simulink model "implfb_can_unpack"  (R2026b)
settings: Solver=VariableStepAuto
undefined symbols (not defined in the file or in its folder): Ts
libraries: simulink x4, svdutilitieslib x1
settings Model: Creator=aomar  LastModifiedBy=aomar

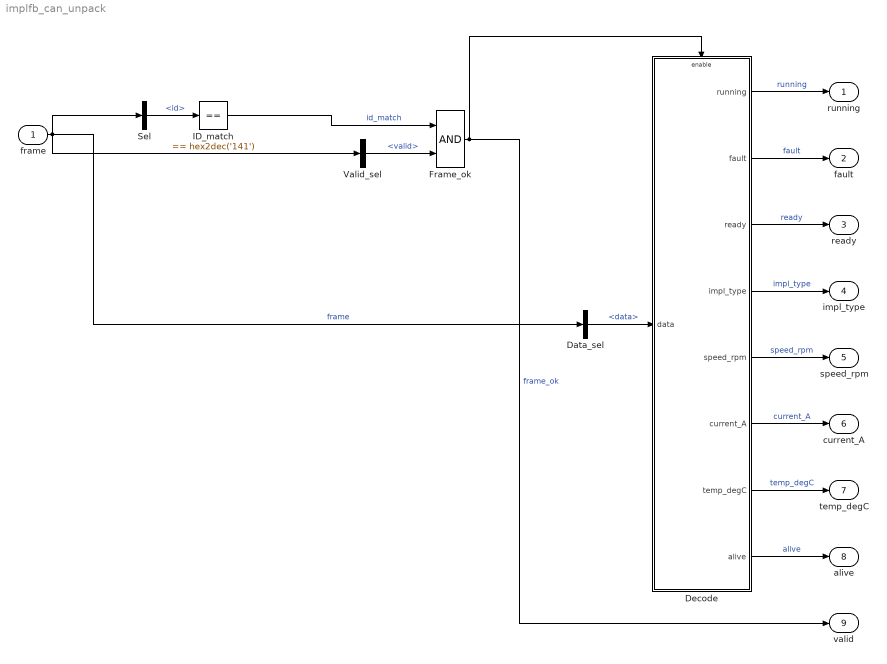
== system implfb_can_unpack ==
  frame : Inport  OutDataTypeStr=Bus: Bus_CanFrame8  SampleTime=Ts.can_slow
  Data_sel : BusSelector  OutputSignals=data
  Decode : Subsystem  TreatAsAtomicUnit=on
  Frame_ok : Logic  AllPortsSameDT=off  OutDataTypeStr=boolean
  ID_match : simulink/Logic and Bit Operations/Compare To Constant  relop===  const=hex2dec('141')  OutDataTypeStr=boolean
  Sel : BusSelector  OutputSignals=id
  Valid_sel : BusSelector  OutputSignals=valid
  running : Outport
  fault : Outport  Port=2
  ready : Outport  Port=3
  impl_type : Outport  Port=4
  speed_rpm : Outport  Port=5
  current_A : Outport  Port=6
  temp_degC : Outport  Port=7
  alive : Outport  Port=8
  valid : Outport  Port=9  OutDataTypeStr=boolean
  wires:
  frame/1 -> Data_sel/1, Sel/1, Valid_sel/1  "frame"
  Sel/1 -> ID_match/1  "<id>"
  ID_match/1 -> Frame_ok/1  "id_match"
  Valid_sel/1 -> Frame_ok/2  "<valid>"
  Frame_ok/1 -> valid/1, Decode/Enable  "frame_ok"
  Data_sel/1 -> Decode/1(data)  "<data>"
  Decode/1(running) -> running/1  "running"
  Decode/2(fault) -> fault/1  "fault"
  Decode/3(ready) -> ready/1  "ready"
  Decode/4(impl_type) -> impl_type/1  "impl_type"
  Decode/5(speed_rpm) -> speed_rpm/1  "speed_rpm"
  Decode/6(current_A) -> current_A/1  "current_A"
  Decode/7(temp_degC) -> temp_degC/1  "temp_degC"
  Decode/8(alive) -> alive/1  "alive"

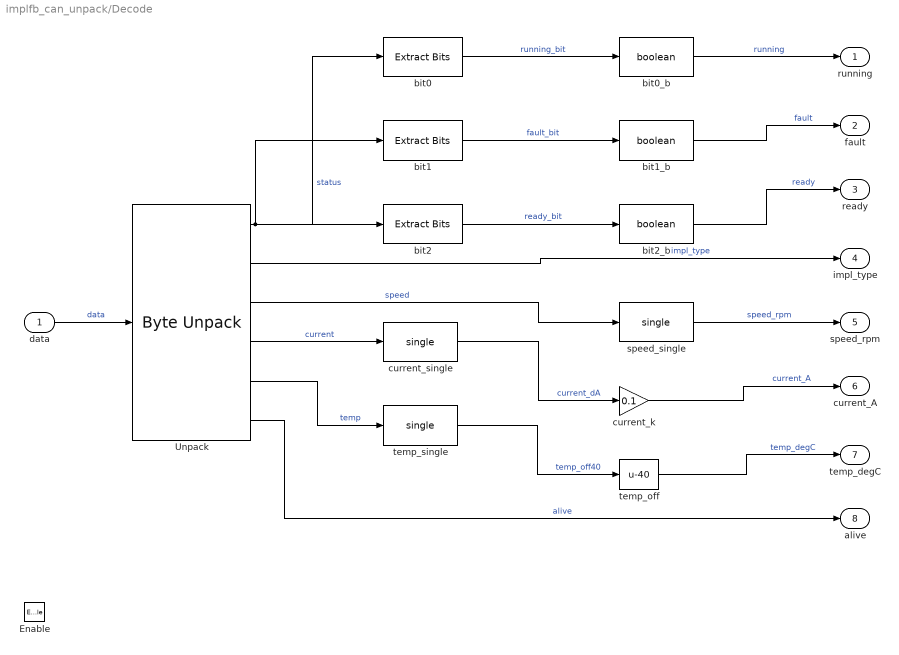
== system implfb_can_unpack/Decode ==
  data : Inport
  Enable : EnablePort
  Unpack : svdutilitieslib/Byte Unpack  dimensions={1,1,1,1,1,1}  datatypes={'uint8','uint8','int16','int16','uint8','uint8'}  byteAlign=1  blockPlatform=arduinoert
      settings: LibrarySourceBlock=mcblib/Signal Management/Byte Unpack
  bit0 : simulink/Logic and Bit Operations/Extract Bits  bitsToExtract=Range of bits  numBits=8  bitIdxRange=[0 0]  outScalingMode=Treat bit field as an integer
  bit0_b : DataTypeConversion  OutDataTypeStr=boolean  RndMeth=Nearest
  bit1 : simulink/Logic and Bit Operations/Extract Bits  bitsToExtract=Range of bits  numBits=8  bitIdxRange=[1 1]  outScalingMode=Treat bit field as an integer
  bit1_b : DataTypeConversion  OutDataTypeStr=boolean  RndMeth=Nearest
  bit2 : simulink/Logic and Bit Operations/Extract Bits  bitsToExtract=Range of bits  numBits=8  bitIdxRange=[2 2]  outScalingMode=Treat bit field as an integer
  bit2_b : DataTypeConversion  OutDataTypeStr=boolean  RndMeth=Nearest
  current_k : Gain  Gain=0.1
  current_single : DataTypeConversion  OutDataTypeStr=single  RndMeth=Nearest
  speed_single : DataTypeConversion  OutDataTypeStr=single  RndMeth=Nearest
  temp_off : Bias  Bias=-40  SaturateOnIntegerOverflow=off
  temp_single : DataTypeConversion  OutDataTypeStr=single  RndMeth=Nearest
  running : Outport  OutDataTypeStr=boolean  InitialOutput=0
  fault : Outport  Port=2  OutDataTypeStr=boolean  InitialOutput=0
  ready : Outport  Port=3  OutDataTypeStr=boolean  InitialOutput=0
  impl_type : Outport  Port=4  OutDataTypeStr=uint8  InitialOutput=0
  speed_rpm : Outport  Port=5  OutDataTypeStr=single  InitialOutput=0
  current_A : Outport  Port=6  OutDataTypeStr=single  InitialOutput=0
  temp_degC : Outport  Port=7  OutDataTypeStr=single  InitialOutput=0
  alive : Outport  Port=8  OutDataTypeStr=uint8  InitialOutput=0
  wires:
  data/1 -> Unpack/1  "data"
  Unpack/1 -> bit0/1, bit1/1, bit2/1  "status"
  Unpack/2 -> impl_type/1  "impl_type"
  Unpack/3 -> speed_single/1  "speed"
  Unpack/4 -> current_single/1  "current"
  Unpack/5 -> temp_single/1  "temp"
  Unpack/6 -> alive/1  "alive"
  current_single/1 -> current_k/1  "current_dA"
  temp_single/1 -> temp_off/1  "temp_off40"
  bit0/1 -> bit0_b/1  "running_bit"
  bit1/1 -> bit1_b/1  "fault_bit"
  bit2/1 -> bit2_b/1  "ready_bit"
  current_k/1 -> current_A/1  "current_A"
  temp_off/1 -> temp_degC/1  "temp_degC"
  bit0_b/1 -> running/1  "running"
  bit1_b/1 -> fault/1  "fault"
  bit2_b/1 -> ready/1  "ready"
  speed_single/1 -> speed_rpm/1  "speed_rpm"
